simulink model "LabExam5"  (R2024b)
settings: Solver=VariableStepAuto  StartTime=0.0  StopTime=1  RelTol=1e-3
libraries: spsRMSLib x4, spsLinearTransformerLib x3, spsACVoltageSourceLib x2, spsCurrentMeasurementLib x2, eePowerMeasurement x2, spsVoltageMeasurementLib x2, sps_lib x1, spspowerguiLib x1
settings Model: Creator=offic  LastModifiedBy=HP

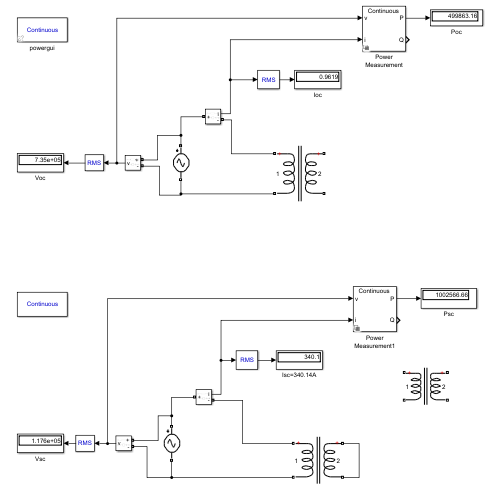
[thumbnail: Simulink's stored preview of the top-level diagram]
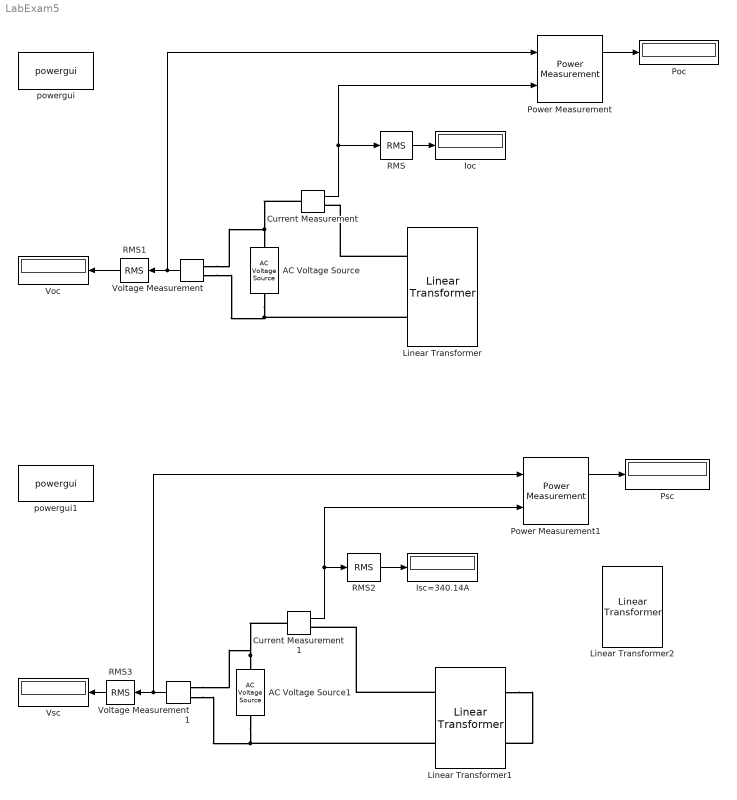
== system LabExam5 ==
  AC Voltage Source : spsACVoltageSourceLib/AC Voltage Source  Amplitude=(7.35e+05)*sqrt(2)  Phase=0  Frequency=60  SampleTime=0  Measurements=None  BusType=swing  Pref=10e3  Qref=0  Qmin=-inf  Qmax=+inf
  AC Voltage Source1 : spsACVoltageSourceLib/AC Voltage Source  Amplitude=(7.35e+05)*sqrt(2)*0.16  Phase=0  Frequency=60  SampleTime=0  Measurements=None  BusType=swing  Pref=10e3  Qref=0  Qmin=-inf  Qmax=+inf
  Current Measurement : spsCurrentMeasurementLib/Current Measurement  PhasorSimulation=off  OutputType=Complex  PSBequivalent=0
  Current Measurement1 : spsCurrentMeasurementLib/Current Measurement  PhasorSimulation=off  OutputType=Complex  PSBequivalent=0
  Ioc : Display
  Isc=340.14A : Display
  Linear Transformer : spsLinearTransformerLib/Linear Transformer  UNITS=SI  NominalPower=[ 250e6 60 ]  winding1=[7.35e+05 4.3218 0.45856]  winding2=[3.15e+05 0.7938 0.084225]  ThreeWindings=off  winding3=[3.15e+05 0.7938 0.084225]  RmLm=[1.0804e+06 2866]  Measurements=None  DataType=on
  Linear Transformer1 : spsLinearTransformerLib/Linear Transformer  UNITS=SI  NominalPower=[ 250e6 60 ]  winding1=[7.35e+05 4.3218 0.45856]  winding2=[3.15e+05 0.7938 0.084225]  ThreeWindings=off  winding3=[3.15e+05 0.7938 0.084225]  RmLm=[1.0804e+06 2866]  Measurements=None  DataType=on
  Linear Transformer2 : spsLinearTransformerLib/Linear Transformer  UNITS=SI  NominalPower=[ 250e6 60 ]  winding1=[7.35e+05 4.3218 0.45856]  winding2=[3.15e+05 0.7938 0.084225]  ThreeWindings=off  winding3=[3.15e+05 0.7938 0.084225]  RmLm=[1.0804e+06 2866]  Measurements=None  DataType=on
  Poc : Display
      settings: Format=bank
  Power Measurement : eePowerMeasurement/Power Measurement  LabelModeActiveChoice=Continuous  F=60  K=[1]  Ts=0
  Power Measurement1 : eePowerMeasurement/Power Measurement  LabelModeActiveChoice=Continuous  F=60  K=[1]  Ts=0
  Psc : Display
      settings: Format=bank
  RMS{,1..3} (4 alike) : spsRMSLib/RMS  TrueRMS=on  Freq=60  RMSInit=120  Ts=0
  Voc : Display
  Voltage Measurement : spsVoltageMeasurementLib/Voltage Measurement  PhasorSimulation=off  OutputType=Complex  PSBequivalent=0
  Voltage Measurement1 : spsVoltageMeasurementLib/Voltage Measurement  PhasorSimulation=off  OutputType=Complex  PSBequivalent=0
  Vsc : Display
  powergui : sps_lib/powergui  Priority=1  SimulationMode=Continuous  SampleTime=50e-6  frequency=60  Iterations=50  frequencyindice=60  Pbase=100e6  ErrMax=1e-4  UnitsV=kV  UnitsW=MW  buscounter=0  FunctionMessages=off  echomessages=off  EnableUseOfTLC=off  CurrentSourceSwitches=off  DisableSnubberDevices=off  DisableRonSwitches=off  DisableVfSwitches=off  DisplayEquations=off  AutomaticDiscreteSolvers=off  SolverType=Tustin/Backward Euler (TBE)  Interpol=off  ExternalGateDelay=off  methode=off  Ts=100  x0status=blocks  SPID=on  SwTol=0  HookPort=off  NonlinearTolerance=1e-4  nMaxIteration=100  ContinueOnMaxIteration=off  RestoreLinks=warning  ResistiveCurrentMeasurement=off  Frange=[0:2:500]  Ylog=off  Xlog=on  ShowGrid=off  save=off  variable=ZData  structure=0  ZoomFFT=off  StartTime=0.0  cycles=1  DisplayStyle=1  fundamental=60  FreqAxis=off  MaxFrequency=1000  frequencyindicesteady=1  RmsSteady=1  display=off
  powergui1 : spspowerguiLib/powergui  Priority=1  SimulationMode=Continuous  SampleTime=50e-6  frequency=60  Iterations=50  frequencyindice=60  Pbase=100e6  ErrMax=1e-4  UnitsV=kV  UnitsW=MW  buscounter=0  FunctionMessages=off  echomessages=off  EnableUseOfTLC=off  CurrentSourceSwitches=off  DisableSnubberDevices=off  DisableRonSwitches=off  DisableVfSwitches=off  DisplayEquations=off  AutomaticDiscreteSolvers=off  SolverType=Tustin/Backward Euler (TBE)  Interpol=off  ExternalGateDelay=off  methode=off  Ts=100  x0status=blocks  SPID=on  SwTol=0  HookPort=off  NonlinearTolerance=1e-4  nMaxIteration=100  ContinueOnMaxIteration=off  RestoreLinks=warning  ResistiveCurrentMeasurement=off  Frange=[0:2:500]  Ylog=off  Xlog=on  ShowGrid=off  save=off  variable=ZData  structure=0  ZoomFFT=off  StartTime=0.0  cycles=1  DisplayStyle=1  fundamental=60  FreqAxis=off  MaxFrequency=1000  frequencyindicesteady=1  RmsSteady=1  display=off
  wires:
  Current Measurement/1 -> Power Measurement/2, RMS/1
  RMS/1 -> Ioc/1
  Voltage Measurement/1 -> Power Measurement/1, RMS1/1
  RMS1/1 -> Voc/1
  Power Measurement/1 -> Poc/1
  RMS3/1 -> Vsc/1
  Power Measurement1/1 -> Psc/1
  Current Measurement1/1 -> Power Measurement1/2, RMS2/1
  RMS2/1 -> Isc=340.14A/1
  Voltage Measurement1/1 -> Power Measurement1/1, RMS3/1
  connections:
  Current Measurement/LConn1 -- Voltage Measurement/LConn1 -- AC Voltage Source/RConn1
  Linear Transformer/LConn1 -- Current Measurement/RConn1
  AC Voltage Source/LConn1 -- Voltage Measurement/LConn2 -- Linear Transformer/LConn2
  AC Voltage Source1/LConn1 -- Linear Transformer1/LConn2 -- Voltage Measurement1/LConn2
  AC Voltage Source1/RConn1 -- Voltage Measurement1/LConn1 -- Current Measurement1/LConn1
  Linear Transformer1/LConn1 -- Current Measurement1/RConn1
  Linear Transformer1/RConn1 -- Linear Transformer1/RConn2
